simulink model "accTracking"  (R2021b)
settings: Solver=VariableStepAuto  StartTime=0.0  StopTime=60  RelTol=1e-3
values from neighbouring files (symbols this model uses):
  g = 32.17405    [SingleDOF.m]    (also in main.m; simio.m = [dx(Index.EOM(1:6)); delta(:)-f; -delta(:)-f ])
  K_lon_hinf = pss(K_lon_hinfs,Domain)    [SingleDOF.m]    (also in main.m)
  LTI_lon = ss(A,B,C,D)    [Dorobantu.m]    (also in mainLinear.m = GTM_lon(:,:,i,j,k); newmain.m = GTM_lon(:,:,i,j,k))
  s = tf('s')    [SingleDOF.m]    (also in main.m; newmain.m)
undefined symbols (not defined in the file or in its folder): ft
libraries: simulink_extras x4, aerolibconvert2 x2
settings Model: Creator=jihoo  LastModifiedBy=jihoo

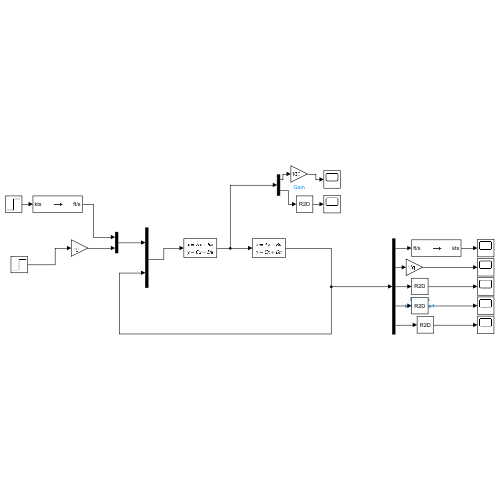
[thumbnail: Simulink's stored preview of the top-level diagram]
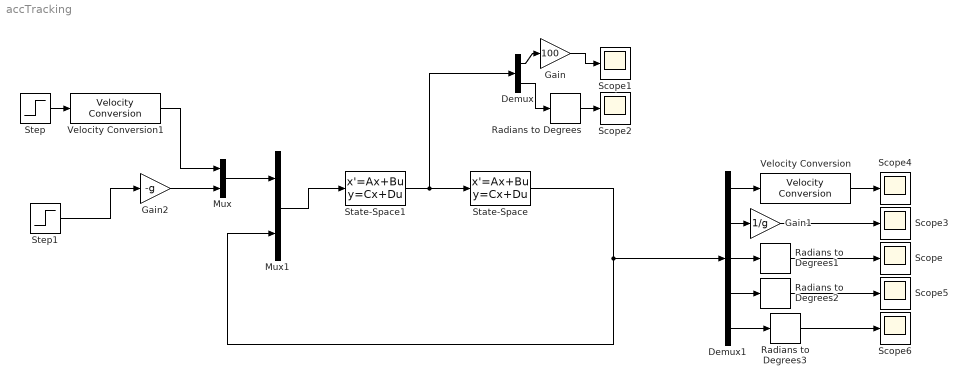
== system accTracking ==
  Demux : Demux  Outputs=2
  Demux1 : Demux  Outputs=5
  Gain : Gain  Gain=100
  Gain1 : Gain  Gain=1/g
  Gain2 : Gain  Gain=-g
  Mux : Mux  Inputs=2
  Mux1 : Mux  Inputs=2
  Radians to Degrees{,1..3} (4 alike) : simulink_extras/Transformations/Radians to Degrees
  Scope{,1..6} (7 alike) : Scope
  State-Space : StateSpace  A=LTI_lon.A  B=LTI_lon.B  C=LTI_lon.C  D=LTI_lon.D  InitialCondition=0
  State-Space1 : StateSpace  A=K_lon_hinf.A  B=K_lon_hinf.B  C=K_lon_hinf.C  D=K_lon_hinf.D  InitialCondition=0
  Step : Step  Time=0  After=10  SampleTime=0
  Step1 : Step  Time=30  SampleTime=0
  Velocity Conversion : aerolibconvert2/Velocity Conversion  IU=ft/s  OU=kts
  Velocity Conversion1 : aerolibconvert2/Velocity Conversion  IU=kts  OU=ft/s
  wires:
  State-Space/1 -> Demux1/1, Mux1/2
  State-Space1/1 -> Demux/1, State-Space/1
  Step/1 -> Velocity Conversion1/1
  Step1/1 -> Gain2/1
  Mux/1 -> Mux1/1
  Mux1/1 -> State-Space1/1
  Radians to Degrees/1 -> Scope2/1
  Demux/2 -> Radians to Degrees/1
  Demux/1 -> Gain/1
  Gain/1 -> Scope1/1
  Demux1/1 -> Velocity Conversion/1
  Demux1/2 -> Gain1/1
  Demux1/3 -> Radians to Degrees1/1
  Demux1/4 -> Radians to Degrees2/1
  Demux1/5 -> Radians to Degrees3/1
  Gain1/1 -> Scope3/1
  Velocity Conversion/1 -> Scope4/1
  Radians to Degrees1/1 -> Scope/1
  Radians to Degrees2/1 -> Scope5/1
  Radians to Degrees3/1 -> Scope6/1
  Gain2/1 -> Mux/2
  Velocity Conversion1/1 -> Mux/1
